simulink model "LR_Model"  (R2024b)
settings: Solver=VariableStepAuto  StartTime=0.0  StopTime=SimulationTime  RelTol=1e-3
values from neighbouring files (symbols this model uses):
  b = 0    [LR_estimation_DCMotor.m]
  J = Jm+Jbl    (= 7.32e-05)    [LR_estimation_DCMotor.m]
  Km = 0.11    [LR_estimation_DCMotor.m]
  L = 4.1e-3    (= 0.0041)    [LR_estimation_DCMotor.m]
  Lstim = cast(Lstim,"double")    [LR_estimation_DCMotor.m]
  R = 3.2    [LR_estimation_DCMotor.m]
  RadToRpm = 60/(2*pi)    (= 9.54929658551)    [LR_estimation_DCMotor.m]
  Rstim = cast(Rstim,"double")    [LR_estimation_DCMotor.m]
  TSample = 0.0001    [LR_estimation_DCMotor.m]
settings Model: Creator=Davide  LastModifiedBy=leonardo.lodolini
settings DataIOCC: ReturnWorkspaceOutputs=off
settings OptimizationCC: ReuseModelBlockBuffer=off
settings RTWCC: GPUComputeCapability=3.5

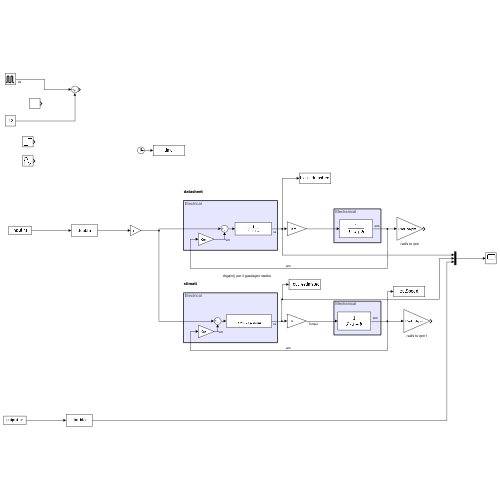
[thumbnail: Simulink's stored preview of the top-level diagram]
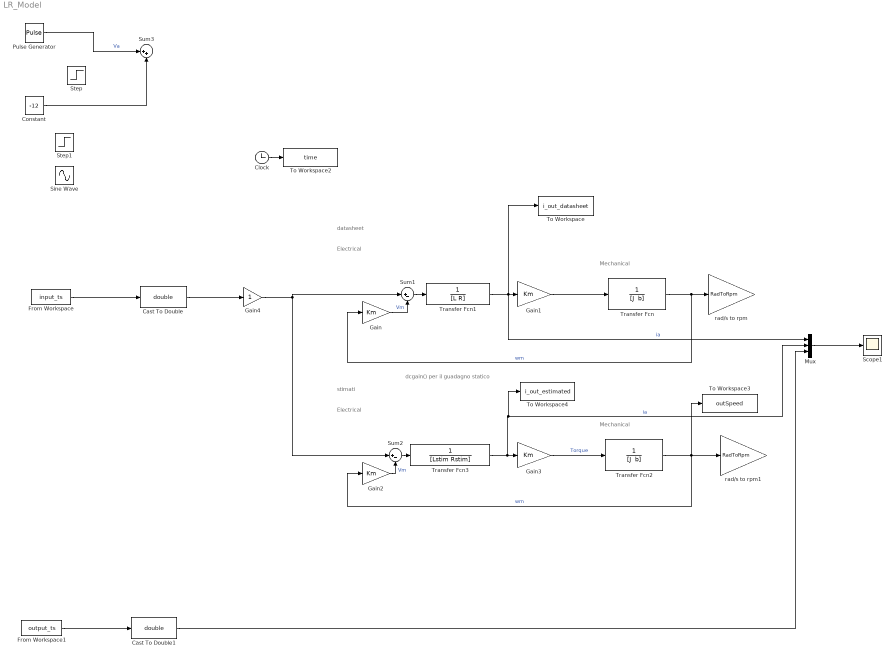
== system LR_Model ==
  note: datasheet
  note: dcgain() per il guadagno statico
  note: Electrical
  note: Mechanical
  note: Electrical
  note: Mechanical
  note: stimati
  Cast To Double : DataTypeConversion  OutDataTypeStr=double  SaturateOnIntegerOverflow=off  RndMeth=Floor
  Cast To Double1 : DataTypeConversion  OutDataTypeStr=double  SaturateOnIntegerOverflow=off  RndMeth=Floor
  Clock : Clock
  Constant : Constant  Value=-12
  From Workspace : FromWorkspace  VariableName=input_ts  SampleTime=TSample
  From Workspace1 : FromWorkspace  VariableName=output_ts  SampleTime=TSample
  Gain{,1..3} (4 alike) : Gain  Gain=Km
  Gain4 : Gain
  Mux : Mux  Inputs=3
  Pulse Generator : DiscretePulseGenerator  PulseType=Time based  Amplitude=24  Period=1  PulseWidth=20  PhaseDelay=-0.002
  Scope1 : Scope
  Sine Wave : Sin  Amplitude=12  Frequency=150  SampleTime=0
  Step : Step  Time=0  After=24  SampleTime=TSample
  Step1 : Step  Time=0  After=24  SampleTime=TSample
  Sum1 : Sum  Inputs=|+-
  Sum2 : Sum  Inputs=|+-
  Sum3 : Sum  Inputs=|++
  To Workspace : ToWorkspace  VariableName=i_out_datasheet  SampleTime=TSample
  To Workspace2 : ToWorkspace  VariableName=time  SampleTime=TSample
  To Workspace3 : ToWorkspace  VariableName=outSpeed  SampleTime=TSample
  To Workspace4 : ToWorkspace  VariableName=i_out_estimated  SampleTime=TSample
  Transfer Fcn : TransferFcn  Denominator="[J  b]"
  Transfer Fcn1 : TransferFcn  Denominator=[L R]
  Transfer Fcn2 : TransferFcn  Denominator="[J  b]"
  Transfer Fcn3 : TransferFcn  Denominator=[Lstim Rstim]
  rad/s to rpm : Gain  Gain=RadToRpm  SaturateOnIntegerOverflow=on  OutDataTypeStr=Inherit: Same as input  ParamDataTypeStr=Inherit: Same as input
  rad/s to rpm1 : Gain  Gain=RadToRpm  SaturateOnIntegerOverflow=on  OutDataTypeStr=Inherit: Same as input  ParamDataTypeStr=Inherit: Same as input
  wires:
  Transfer Fcn/1 -> rad/s to rpm/1, Gain/1  "wm"
  Transfer Fcn1/1 -> Mux/1, To Workspace/1, Gain1/1  "ia"
  Sum1/1 -> Transfer Fcn1/1
  Gain/1 -> Sum1/2  "Vm"
  Sum2/1 -> Transfer Fcn3/1
  Gain3/1 -> Transfer Fcn2/1  "Torque"
  Transfer Fcn3/1 -> To Workspace4/1, Mux/2, Gain3/1  "ia"
  Transfer Fcn2/1 -> To Workspace3/1, Gain2/1, rad/s to rpm1/1  "wm"
  Gain2/1 -> Sum2/2  "Vm"
  Mux/1 -> Scope1/1
  Gain1/1 -> Transfer Fcn/1
  Clock/1 -> To Workspace2/1
  Constant/1 -> Sum3/2
  From Workspace/1 -> Cast To Double/1
  Pulse Generator/1 -> Sum3/1  "Va"
  Gain4/1 -> Sum2/1, Sum1/1
  Cast To Double/1 -> Gain4/1
  From Workspace1/1 -> Cast To Double1/1
  Cast To Double1/1 -> Mux/3
